simulink model "Flight3Dof_V"  (R2024b)
settings: Solver=VariableStepAuto  StartTime=0.0  StopTime=90
values from neighbouring files (symbols this model uses):
  alpha_sch = [0 0.08 0.16 0.24 0.32 0.4]    [aero_guid_autop.mat]
  Cm_q = -0.65    [aero_guid_dat.m]
  Cn_alpha = 7.609    [aero_guid_dat.m]
  Cx_fin = 0    [aero_guid_dat.m]
  Cz_fin = 5.61    [aero_guid_dat.m]
  d_ref = 0.08    [aero_guid_dat.m]
  fin_max = 35.0*d2r    (= 0.610865238198)    [aero_guid_dat.m]
  fin_min = -35.0*d2r    (= -0.610865238198)    [aero_guid_dat.m]
  g = 9.81    [aero_guid_dat.m]
  h_ini = mState(end,4)    [aero_guid_dat.m]
  K = [0.0274272658442 0.022514521532 0.0188381278441 0.0160368406712 0.0137662609944 0.0119857576445 0.0105918197111 0.00938210037551 0.00839164223299 0.0264249961464 0.0216246329404 0.0181908758086 ... (54 elements, 9x6)]    [aero_guid_autop.mat]
  Ka = [0.941240537955 0.93637246732 0.931559594469 0.926913222355 0.921953565217 0.917255055328 0.913053581223 0.908386604457 0.903975208808 0.938862932336 0.933592325749 0.928951336073 ... (54 elements, 9x6)]    [aero_guid_autop.mat]
  Kg = [0.85025548389 0.668816232249 0.539692221599 0.444760785577 0.373115794158 0.317881150033 0.273934317038 0.239434726051 0.211636994858 0.843001258735 0.661554199177 0.532424138805 ... (54 elements, 9x6)]    [aero_guid_autop.mat]
  Ki = [22.5219818693 26.1087313803 30.1256514292 34.5615685684 39.3998846557 44.6135139259 50.5273670311 56.4127258892 62.5431134445 22.709249563 26.3788303432 30.5068602639 ... (54 elements, 9x6)]    [aero_guid_autop.mat]
  l_acc = 0.07465    [aero_guid_dat.m]
  M_sch = [0 0.25 0.5 0.75 1 1.25 1.5 1.75 2]    [aero_guid_autop.mat]
  max_acc = max_load_factor*g    (= 58.86)    [aero_guid_dat.m]
  pos_tgt = [x_ini_tgt,-h_ini_tgt]    [aero_guid_dat.m]
  q_ini = 0.00001*d2r    (= 1.74532925199e-07)    [aero_guid_dat.m]
  S_ref = 0.0050    (= 0.005)    [aero_guid_dat.m]
  t_fin_burn = 30    [aero_guid_dat.m]
  theta_tgt = 180*d2r    (= 3.14159265359)    [aero_guid_dat.m]
  Thrust = 150    [aero_guid_dat.m]
  v_ini = sqrt(mState(end,1)^2+mState(end,2)^2)    [aero_guid_dat.m]
  v_tgt = 60    [aero_guid_dat.m]
  X_cp = 0.6873    [aero_guid_dat.m]
  x_ini = mState(end,3)    [aero_guid_dat.m]
undefined symbols (not defined in the file or in its folder): CG_with_time, Cx_with_M, mass_with_time, mdot, Pk_final, Pk_matrix_small, theta_vec, theta_vec_small, X_cg, X_cg_fixed_small, Y_cg, Y_cg_fixed_small
libraries: aerolibasang x3, simulink x2, aerolibanim x1, aerolibatmos2 x1, aerolibactuator x1
settings Model: Creator=vince  LastModifiedBy=vince
settings SolverCC: ZeroCrossAlgorithm=Adaptive
settings DebuggingCC: AlgebraicLoopMsg=none  IgnoredZcDiagnostic=none
settings RTWCC: GPUComputeCapability=3.5

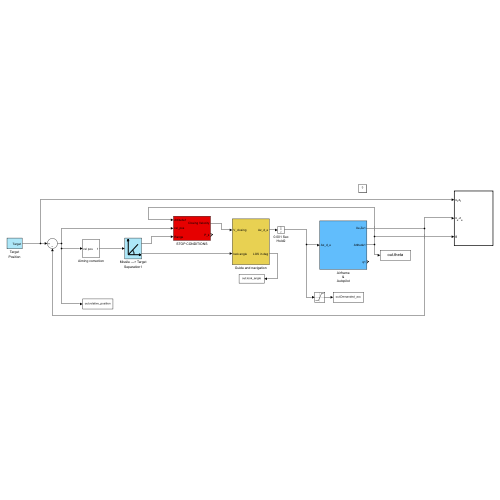
[thumbnail: Simulink's stored preview of the top-level diagram]
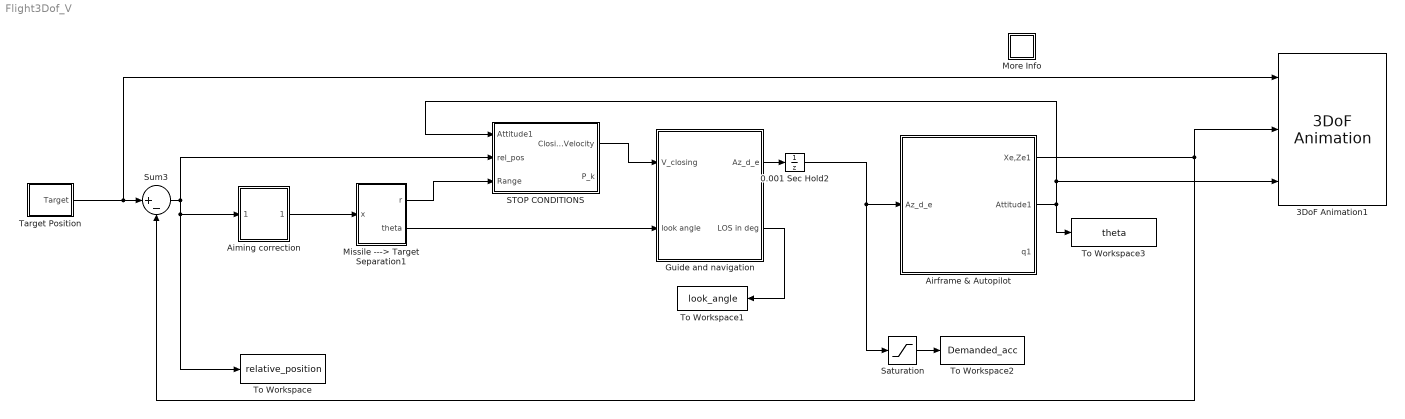
== system Flight3Dof_V ==
  0.001 Sec Hold2 : UnitDelay  SampleTime=0.001  HasFrameUpgradeWarning=on
  3DoF Animation1 : aerolibanim/3DoF Animation  u1=[0 10000 0 100000 -10000 -50]  u2=0.1  u3=5  u5=Fixed position  u6=[2000 18000 -3150]  u7=10  u8=on
  Aiming correction : Subsystem
  Airframe & Autopilot : Subsystem
  Guide and navigation : Subsystem
  Missile ---> Target Separation1 : Subsystem  mask(Cart2Polar){}
      mask help:
      | Transformation from cartesian to polar coordinates.
      | [x, y] -> [r, theta]
      |
      | r = sqrt(x^2 + y^2);
      | theta = atan(y/x);
      mask Help: Unmask this block for more help.
      mask Display: plot(0,0,100,100,[24,20,15,20,20],[85,95,85,95,20],[80,20,95,85,95,85],[70,20,20,15,20,24],[56,56,55,52,50,46],[20,26,31,35,38,42])
  More Info : Subsystem
      settings: OpenFcn=showExample('simulink_aerospace/DesigningAGuidanceSystemInMATLABAndSimulinkExample')
      mask Display: disp('?')
  STOP CONDITIONS : Subsystem
  Saturation : Saturate  UpperLimit=max_acc  LowerLimit=-max_acc
  Sum3 : Sum  Inputs=|+-  InputSameDT=on  SaturateOnIntegerOverflow=on  OutDataTypeStr=Inherit: Same as first input
  Target Position : Subsystem
  To Workspace : ToWorkspace  VariableName=relative_position  SampleTime=-1
  To Workspace1 : ToWorkspace  VariableName=look_angle  SaveFormat=Structure With Time  SampleTime=-1
  To Workspace2 : ToWorkspace  VariableName=Demanded_acc  SaveFormat=Structure With Time  SampleTime=-1
  To Workspace3 : ToWorkspace  VariableName=theta  SaveFormat=Structure With Time  SampleTime=-1
  wires:
  Sum3/1 -> To Workspace/1, Aiming correction/1(rel pos), STOP CONDITIONS/2(rel_pos)
  Target Position/1(Target) -> 3DoF Animation1/1, Sum3/1
  Airframe & Autopilot/1(Xe,Ze1) -> Sum3/2, 3DoF Animation1/2
  Airframe & Autopilot/2(Attitude1) -> To Workspace3/1, STOP CONDITIONS/1(Attitude1), 3DoF Animation1/3
  Guide and navigation/1(Az_d_e) -> 0.001 Sec Hold2/1
  Missile ---> Target Separation1/2(theta) -> Guide and navigation/2(look angle)
  Guide and navigation/2(LOS in deg) -> To Workspace1/1
  STOP CONDITIONS/1(Closing Velocity) -> Guide and navigation/1(V_closing)
  Missile ---> Target Separation1/1(r) -> STOP CONDITIONS/3(Range)
  Aiming correction/1(Out1) -> Missile ---> Target Separation1/1(x)
  0.001 Sec Hold2/1 -> Saturation/1, Airframe & Autopilot/1(Az_d_e)
  Saturation/1 -> To Workspace2/1

== system Flight3Dof_V/Aiming correction ==
  rel pos : Inport
  Add : Sum
  Add1 : Sum
  Demux1 : Demux  Outputs=2
  Mux : Mux  Inputs=2
  x error : Constant  Value=0.6
  z error : Constant  Value=0.65
  Out1 : Outport
  wires:
  rel pos/1 -> Demux1/1
  Demux1/2 -> Add1/1
  Demux1/1 -> Add/2
  Mux/1 -> Out1/1
  Add/1 -> Mux/1
  x error/1 -> Add/1
  Add1/1 -> Mux/2
  z error/1 -> Add1/2

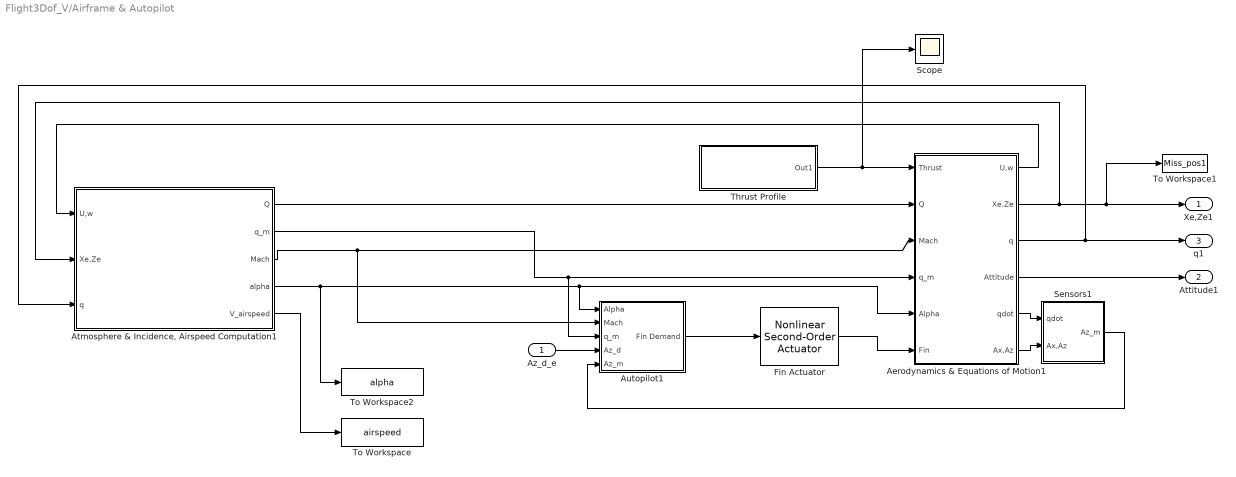
== system Flight3Dof_V/Airframe & Autopilot ==
  Az_d_e : Inport
  Aerodynamics & Equations of Motion1 : Subsystem
  "Atmosphere & Incidence, Airspeed Computation1" : Subsystem
  Autopilot1 : Subsystem
  Fin Actuator : aerolibactuator/Nonlinear Second-Order Actuator  wn_fin=wn_fin  z_fin=z_fin  fin_max=fin_max  fin_min=fin_min  fin_maxrate=fin_maxrate  fin_act_0=fin_act_0  fin_act_vel=0
  Scope : Scope
  Sensors1 : Subsystem
  Thrust Profile : Subsystem
  To Workspace : ToWorkspace  VariableName=airspeed  SaveFormat=Structure With Time  SampleTime=-1
  To Workspace1 : ToWorkspace  VariableName=Miss_pos1  SaveFormat=Structure With Time  SampleTime=-1
  To Workspace2 : ToWorkspace  VariableName=alpha  SaveFormat=Structure With Time  SampleTime=-1
  Xe,Ze1 : Outport  InitialOutput=0  VectorParamsAs1DForOutWhenUnconnected=off
  Attitude1 : Outport  Port=2  InitialOutput=0  VectorParamsAs1DForOutWhenUnconnected=off
  q1 : Outport  Port=3  InitialOutput=0  VectorParamsAs1DForOutWhenUnconnected=off
  wires:
  "Atmosphere & Incidence, Airspeed Computation1"/4(alpha) -> Autopilot1/1(Alpha), Aerodynamics & Equations of Motion1/5(Alpha), To Workspace2/1
  Aerodynamics & Equations of Motion1/3(q) -> "Atmosphere & Incidence, Airspeed Computation1"/3(q), q1/1
  "Atmosphere & Incidence, Airspeed Computation1"/2(q_m) -> Autopilot1/3(q_m), Aerodynamics & Equations of Motion1/4(q_m)
  "Atmosphere & Incidence, Airspeed Computation1"/1(Q) -> Aerodynamics & Equations of Motion1/2(Q)
  Aerodynamics & Equations of Motion1/4(Attitude) -> Attitude1/1
  Aerodynamics & Equations of Motion1/1(U,w) -> "Atmosphere & Incidence, Airspeed Computation1"/1(U,w)
  Aerodynamics & Equations of Motion1/2(Xe,Ze) -> "Atmosphere & Incidence, Airspeed Computation1"/2(Xe,Ze), To Workspace1/1, Xe,Ze1/1
  Aerodynamics & Equations of Motion1/6(Ax,Az) -> Sensors1/2(Ax,Az)
  Aerodynamics & Equations of Motion1/5(qdot) -> Sensors1/1(qdot)
  Sensors1/1(Az_m) -> Autopilot1/5(Az_m)
  "Atmosphere & Incidence, Airspeed Computation1"/3(Mach) -> Autopilot1/2(Mach), Aerodynamics & Equations of Motion1/3(Mach)
  "Atmosphere & Incidence, Airspeed Computation1"/5(V_airspeed) -> To Workspace/1
  Thrust Profile/1(Out1) -> Scope/1, Aerodynamics & Equations of Motion1/1(Thrust)
  Fin Actuator/1 -> Aerodynamics & Equations of Motion1/6(Fin)
  Az_d_e/1 -> Autopilot1/4(Az_d)
  Autopilot1/1(Fin Demand) -> Fin Actuator/1

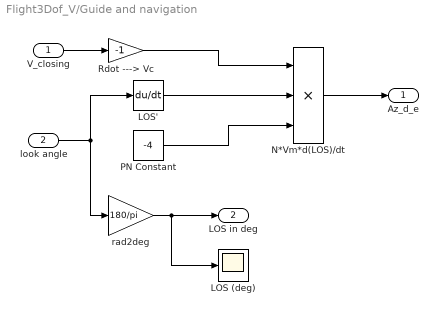
== system Flight3Dof_V/Guide and navigation ==
  V_closing : Inport
  look angle : Inport  Port=2
  LOS (deg) : Scope
  LOS' : Derivative
  N*Vm*d(LOS)/dt : Product  Inputs=3
  PN Constant : Constant  Value=-4
  Rdot ---> Vc : Gain  Gain=-1  SaturateOnIntegerOverflow=on  OutDataTypeStr=Inherit: Same as input  ParamDataTypeStr=Inherit: Same as input
  rad2deg : Gain  Gain=180/pi
  Az_d_e : Outport
  LOS in deg : Outport  Port=2
  wires:
  LOS'/1 -> N*Vm*d(LOS)/dt/2
  rad2deg/1 -> LOS (deg)/1, LOS in deg/1
  N*Vm*d(LOS)/dt/1 -> Az_d_e/1
  look angle/1 -> LOS'/1, rad2deg/1
  V_closing/1 -> Rdot ---> Vc/1
  PN Constant/1 -> N*Vm*d(LOS)/dt/3
  Rdot ---> Vc/1 -> N*Vm*d(LOS)/dt/1

== system Flight3Dof_V/Missile ---> Target Separation1 ==
  x : Inport
  Range : Fcn  Expr=hypot(u[1],u[2])
  Sightline Angle : Fcn  Expr=atan2(-u[2],u[1])
  r : Outport  InitialOutput=0  VectorParamsAs1DForOutWhenUnconnected=off
  theta : Outport  Port=2  InitialOutput=0  VectorParamsAs1DForOutWhenUnconnected=off
  wires:
  x/1 -> Sightline Angle/1, Range/1
  Range/1 -> r/1
  Sightline Angle/1 -> theta/1

== system Flight3Dof_V/More Info ==

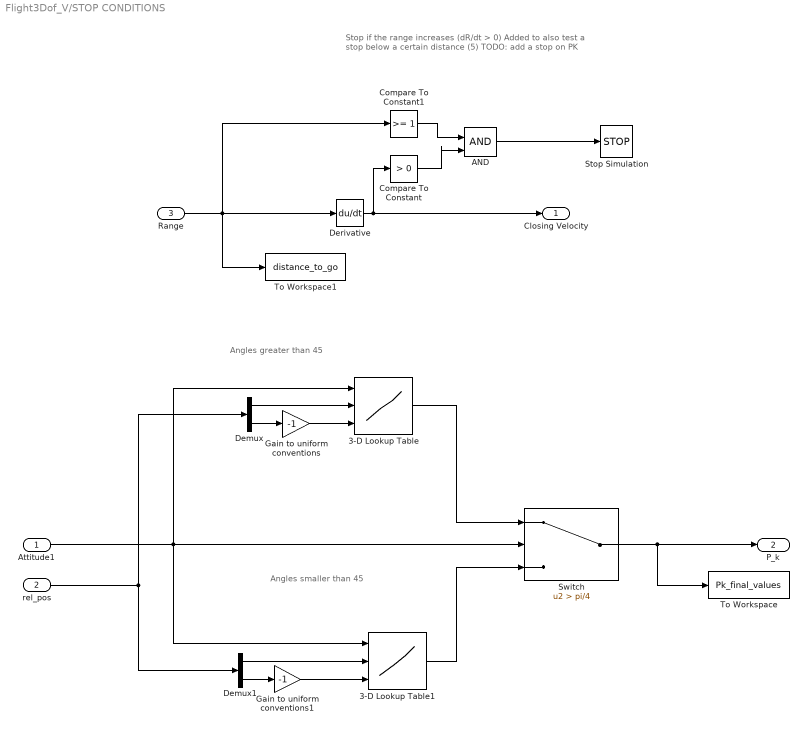
== system Flight3Dof_V/STOP CONDITIONS ==
  note: Angles greater than 45
  note: Stop if the range increases (dR/dt > 0)
      |
      | Added to also test a stop below a certain distance (5)
      |
      | TODO: add a stop on PK
  note: Angles smaller than 45
  Attitude1 : Inport
  rel_pos : Inport  Port=2
  Range : Inport  Port=3
  3-D Lookup Table : Lookup_n-D  NumberOfTableDimensions=3  BreakpointsForDimension1=theta_vec  BreakpointsForDimension2=X_cg  BreakpointsForDimension3=Y_cg  Table=Pk_final  ExtrapMethod=Clip  InternalRulePriority=Speed  RndMeth=Simplest
      settings: InputPortMap=u0,u1,u2
  3-D Lookup Table1 : Lookup_n-D  NumberOfTableDimensions=3  BreakpointsForDimension1=theta_vec_small  BreakpointsForDimension2=X_cg_fixed_small  BreakpointsForDimension3=Y_cg_fixed_small  Table=Pk_matrix_small  ExtrapMethod=Clip  InternalRulePriority=Speed  RndMeth=Simplest
      settings: InputPortMap=u0,u1,u2
  AND : Logic  IconShape=distinctive  AllPortsSameDT=off  OutDataTypeStr=boolean
  Compare To Constant : simulink/Logic and Bit Operations/Compare To Constant  relop=>  const=0  OutDataTypeStr=boolean
  Compare To Constant1 : simulink/Logic and Bit Operations/Compare To Constant  relop=>=  const=1  OutDataTypeStr=boolean
  Demux : Demux  Outputs=2
  Demux1 : Demux  Outputs=2
  Derivative : Derivative
  Gain to uniform conventions : Gain  Gain=-1
  Gain to uniform conventions1 : Gain  Gain=-1
  Stop Simulation : Stop
  Switch : Switch  Criteria=u2 > Threshold  Threshold=pi/4  SaturateOnIntegerOverflow=off  InputSameDT=off
  To Workspace : ToWorkspace  VariableName=Pk_final_values  SaveFormat=Structure With Time  SampleTime=-1
  To Workspace1 : ToWorkspace  VariableName=distance_to_go  SaveFormat=Structure With Time  SampleTime=-1
  Closing Velocity : Outport
  P_k : Outport  Port=2
  wires:
  Range/1 -> Compare To Constant1/1, Derivative/1, To Workspace1/1
  Derivative/1 -> Closing Velocity/1, Compare To Constant/1
  rel_pos/1 -> Demux/1, Demux1/1
  3-D Lookup Table/1 -> Switch/1
  Demux/1 -> 3-D Lookup Table/2
  Demux/2 -> Gain to uniform conventions/1
  Gain to uniform conventions/1 -> 3-D Lookup Table/3
  3-D Lookup Table1/1 -> Switch/3
  Demux1/2 -> Gain to uniform conventions1/1
  Demux1/1 -> 3-D Lookup Table1/2
  Attitude1/1 -> 3-D Lookup Table/1, 3-D Lookup Table1/1, Switch/2
  Gain to uniform conventions1/1 -> 3-D Lookup Table1/3
  Switch/1 -> To Workspace/1, P_k/1
  Compare To Constant1/1 -> AND/1
  Compare To Constant/1 -> AND/2
  AND/1 -> Stop Simulation/1

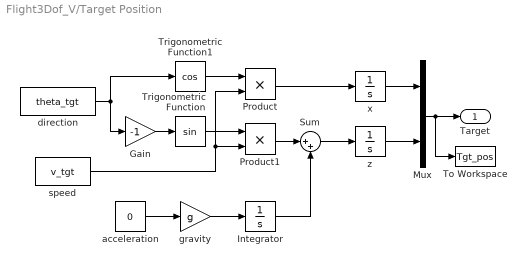
== system Flight3Dof_V/Target Position ==
  Gain : Gain  Gain=-1  SaturateOnIntegerOverflow=on  OutDataTypeStr=Inherit: Same as input  ParamDataTypeStr=Inherit: Same as input
  Integrator : Integrator
  Mux : Mux  Inputs=2
  Product : Product  InputSameDT=on  SaturateOnIntegerOverflow=on  OutDataTypeStr=Inherit: Same as first input
  Product1 : Product  InputSameDT=on  SaturateOnIntegerOverflow=on  OutDataTypeStr=Inherit: Same as first input
  Sum : Sum  Inputs=|++
  To Workspace : ToWorkspace  VariableName=Tgt_pos  SaveFormat=Structure  SampleTime=-1
  Trigonometric Function : Trigonometry
  Trigonometric Function1 : Trigonometry  Operator=cos
  acceleration : Constant  Value=0
  direction : Constant  Value=theta_tgt
  gravity : Gain  Gain=g
  speed : Constant  Value=v_tgt
  x : Integrator  InitialCondition=pos_tgt(1)
  z : Integrator  InitialCondition=pos_tgt(2)
  Target : Outport  VectorParamsAs1DForOutWhenUnconnected=off
  wires:
  x/1 -> Mux/1
  z/1 -> Mux/2
  Product/1 -> x/1
  speed/1 -> Product/2, Product1/2
  Trigonometric Function/1 -> Product1/1
  Trigonometric Function1/1 -> Product/1
  direction/1 -> Trigonometric Function1/1, Gain/1
  Gain/1 -> Trigonometric Function/1
  Mux/1 -> Target/1, To Workspace/1
  Product1/1 -> Sum/1
  Sum/1 -> z/1
  acceleration/1 -> gravity/1
  gravity/1 -> Integrator/1
  Integrator/1 -> Sum/2

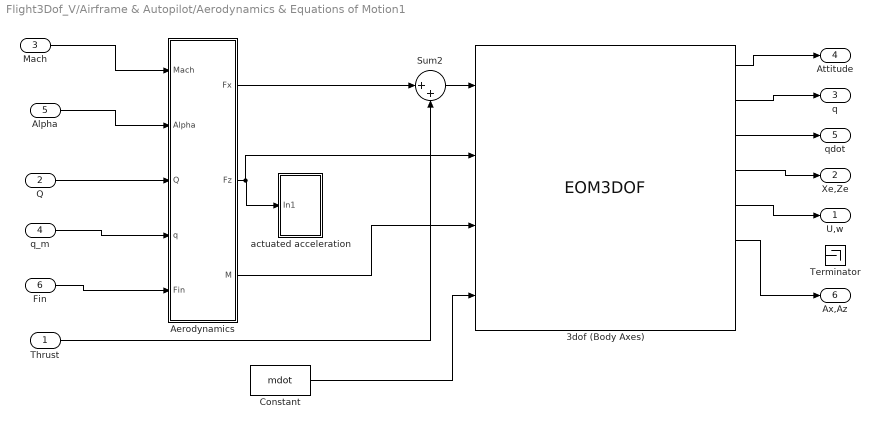
== system Flight3Dof_V/Airframe & Autopilot/Aerodynamics & Equations of Motion1 ==
  Thrust : Inport
  Q : Inport  Port=2
  Mach : Inport  Port=3
  q_m : Inport  Port=4
  Alpha : Inport  Port=5
  Fin : Inport  Port=6
  3dof (Body Axes) : EOM3DOF  mtype=Simple Variable  v_ini=v_ini  theta_ini=theta_ini  q_ini=q_ini  alpha_ini=alpha_ini  pos_ini=[x_ini -h_ini]  mass=mass_full  mass_e=mass_empty  mass_f=mass_full  Iyy=Iyy_full  Iyy_e=Iyy_empty  Iyy_f=Iyy_full  abi_flag=on
  Aerodynamics : Subsystem
  Constant : Constant  Value=mdot
  Sum2 : Sum  Inputs=|++  InputSameDT=on  SaturateOnIntegerOverflow=on  OutDataTypeStr=Inherit: Same as first input
  Terminator : Terminator
  actuated acceleration : Subsystem
  U,w : Outport  InitialOutput=0  VectorParamsAs1DForOutWhenUnconnected=off
  Xe,Ze : Outport  Port=2  InitialOutput=0  VectorParamsAs1DForOutWhenUnconnected=off
  q : Outport  Port=3  InitialOutput=0  VectorParamsAs1DForOutWhenUnconnected=off
  Attitude : Outport  Port=4  InitialOutput=0  VectorParamsAs1DForOutWhenUnconnected=off
  qdot : Outport  Port=5  InitialOutput=0  VectorParamsAs1DForOutWhenUnconnected=off
  Ax,Az : Outport  Port=6  InitialOutput=0  VectorParamsAs1DForOutWhenUnconnected=off
  wires:
  Sum2/1 -> 3dof (Body Axes)/1
  Aerodynamics/1(Fx) -> Sum2/1
  Thrust/1 -> Sum2/2
  q_m/1 -> Aerodynamics/4(q)
  Q/1 -> Aerodynamics/3(Q)
  Alpha/1 -> Aerodynamics/2(Alpha)
  3dof (Body Axes)/6 -> Ax,Az/1
  3dof (Body Axes)/5 -> U,w/1
  3dof (Body Axes)/4 -> Xe,Ze/1
  3dof (Body Axes)/3 -> qdot/1
  3dof (Body Axes)/2 -> q/1
  3dof (Body Axes)/1 -> Attitude/1
  Constant/1 -> 3dof (Body Axes)/4
  Aerodynamics/2(Fz) -> 3dof (Body Axes)/2, actuated acceleration/1(In1)
  Aerodynamics/3(" M") -> 3dof (Body Axes)/3
  Fin/1 -> Aerodynamics/5(Fin)
  Mach/1 -> Aerodynamics/1(Mach)

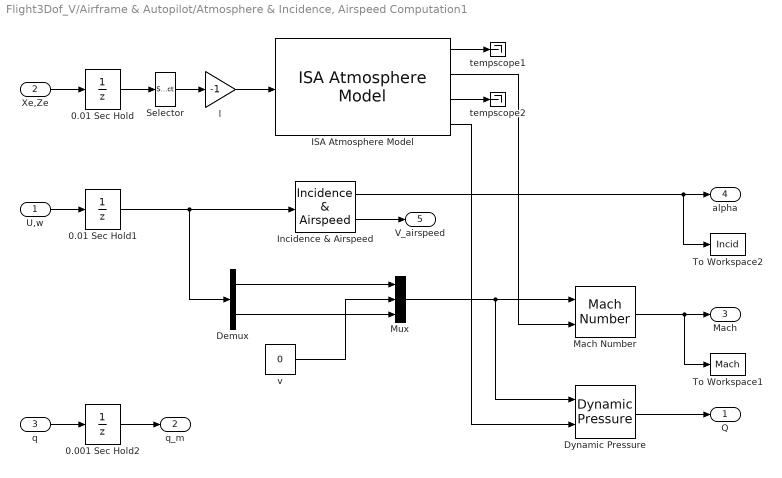
== system Flight3Dof_V/Airframe & Autopilot/Atmosphere & Incidence, Airspeed Computation1 ==
  U,w : Inport
  Xe,Ze : Inport  Port=2
  q : Inport  Port=3
  0.001 Sec Hold2 : UnitDelay  InitialCondition=q_ini  SampleTime=0.001  HasFrameUpgradeWarning=on
  0.01 Sec Hold : UnitDelay  InitialCondition=[x_ini -h_ini]  SampleTime=0.01  HasFrameUpgradeWarning=on
  0.01 Sec Hold1 : UnitDelay  InitialCondition=[v_ini 0]  SampleTime=0.01  HasFrameUpgradeWarning=on
  Demux : Demux  Outputs=2
  Dynamic Pressure : aerolibasang/Dynamic Pressure
  ISA Atmosphere Model : aerolibatmos2/ISA Atmosphere Model  useExtended=off  action=Warning  custom=off  viscosityOut=off  g=9.80665  gamma=1.4  R=287.0531  L=0.0065  h_trop=11000  h_strat=20000  rho0=1.225  P0=101325  T0=288.15  h0=0  S=110.4  Tref=273.15  muref=1.716e-5
  Incidence & Airspeed : aerolibasang/Incidence  & Airspeed
  Mach Number : aerolibasang/Mach Number
  Mux : Mux  Inputs=3
  Selector : Selector  InputPortWidth=2  IndexOptions=Index vector (dialog)  Indices=[2]  OutputSizes=1
  To Workspace1 : ToWorkspace  VariableName=Mach  SaveFormat=Structure With Time  SampleTime=-1
  To Workspace2 : ToWorkspace  VariableName=Incid  SaveFormat=Structure With Time  SampleTime=-1
  l : Gain  Gain=-1  SaturateOnIntegerOverflow=on  OutDataTypeStr=Inherit: Same as input  ParamDataTypeStr=Inherit: Same as input
  tempscope1 : Terminator
  tempscope2 : Terminator
  v : Constant  Value=0
  Q : Outport
  q_m : Outport  Port=2
  Mach : Outport  Port=3
  alpha : Outport  Port=4
  V_airspeed : Outport  Port=5
  wires:
  U,w/1 -> 0.01 Sec Hold1/1
  Incidence & Airspeed/1 -> To Workspace2/1, alpha/1
  Demux/1 -> Mux/1
  Demux/2 -> Mux/3
  v/1 -> Mux/2
  Mux/1 -> Mach Number/1, Dynamic Pressure/1
  Incidence & Airspeed/2 -> V_airspeed/1
  ISA Atmosphere Model/4 -> Dynamic Pressure/2
  Mach Number/1 -> To Workspace1/1, Mach/1
  Dynamic Pressure/1 -> Q/1
  0.01 Sec Hold1/1 -> Incidence & Airspeed/1, Demux/1
  0.01 Sec Hold/1 -> Selector/1
  l/1 -> ISA Atmosphere Model/1
  ISA Atmosphere Model/1 -> tempscope1/1
  ISA Atmosphere Model/3 -> tempscope2/1
  Selector/1 -> l/1
  Xe,Ze/1 -> 0.01 Sec Hold/1
  ISA Atmosphere Model/2 -> Mach Number/2
  0.001 Sec Hold2/1 -> q_m/1
  q/1 -> 0.001 Sec Hold2/1

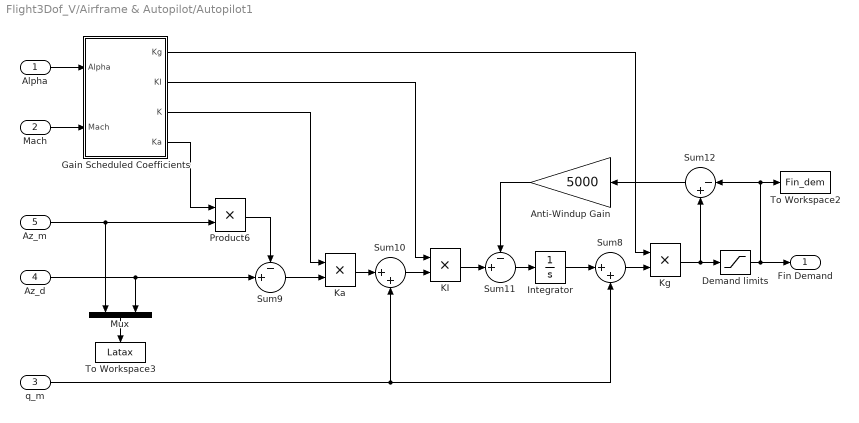
== system Flight3Dof_V/Airframe & Autopilot/Autopilot1 ==
  Alpha : Inport
  Mach : Inport  Port=2
  q_m : Inport  Port=3
  Az_d : Inport  Port=4
  Az_m : Inport  Port=5
  Anti-Windup Gain : Gain  Gain=5000  SaturateOnIntegerOverflow=on  OutDataTypeStr=Inherit: Same as input  ParamDataTypeStr=Inherit: Same as input
  "Demand limits " : Saturate  UpperLimit=fin_max  LowerLimit=fin_min
  Gain Scheduled Coefficients : Subsystem
  Integrator : Integrator
  KI : Product  InputSameDT=on  SaturateOnIntegerOverflow=on  OutDataTypeStr=Inherit: Same as first input
  Ka : Product  InputSameDT=on  SaturateOnIntegerOverflow=on  OutDataTypeStr=Inherit: Same as first input
  Kg : Product  InputSameDT=on  SaturateOnIntegerOverflow=on  OutDataTypeStr=Inherit: Same as first input
  Mux : Mux  Inputs=2
  Product6 : Product  InputSameDT=on  SaturateOnIntegerOverflow=on  OutDataTypeStr=Inherit: Same as first input
  Sum10 : Sum  Inputs=|++  InputSameDT=on  SaturateOnIntegerOverflow=on  OutDataTypeStr=Inherit: Same as first input
  Sum11 : Sum  Inputs=-+|  InputSameDT=on  SaturateOnIntegerOverflow=on  OutDataTypeStr=Inherit: Same as first input
  Sum12 : Sum  Inputs=|-+  InputSameDT=on  SaturateOnIntegerOverflow=on  OutDataTypeStr=Inherit: Same as first input
  Sum8 : Sum  Inputs=|++  InputSameDT=on  SaturateOnIntegerOverflow=on  OutDataTypeStr=Inherit: Same as first input
  Sum9 : Sum  Inputs=-+|  InputSameDT=on  SaturateOnIntegerOverflow=on  OutDataTypeStr=Inherit: Same as first input
  To Workspace2 : ToWorkspace  VariableName=Fin_dem  SaveFormat=Structure With Time  SampleTime=-1
  To Workspace3 : ToWorkspace  VariableName=Latax  SaveFormat=Structure With Time  SampleTime=-1
  Fin Demand : Outport  InitialOutput=0  VectorParamsAs1DForOutWhenUnconnected=off
  wires:
  Mach/1 -> Gain Scheduled Coefficients/2(Mach)
  Alpha/1 -> Gain Scheduled Coefficients/1(Alpha)
  Kg/1 -> Sum12/2, "Demand limits "/1
  Gain Scheduled Coefficients/1("Kg ") -> Kg/1
  Gain Scheduled Coefficients/3("K ") -> Ka/1
  Gain Scheduled Coefficients/2("KI ") -> KI/1
  Anti-Windup Gain/1 -> Sum11/1
  Sum8/1 -> Kg/2
  Integrator/1 -> Sum8/1
  Sum11/1 -> Integrator/1
  Product6/1 -> Sum9/1
  Sum9/1 -> Ka/2
  Ka/1 -> Sum10/1
  Sum10/1 -> KI/2
  KI/1 -> Sum11/2
  Sum12/1 -> Anti-Windup Gain/1
  Az_d/1 -> Mux/2, Sum9/2
  Mux/1 -> To Workspace3/1
  q_m/1 -> Sum10/2, Sum8/2
  "Demand limits "/1 -> Fin Demand/1, Sum12/1, To Workspace2/1
  Az_m/1 -> Mux/1, Product6/2
  Gain Scheduled Coefficients/4("Ka ") -> Product6/1

== system Flight3Dof_V/Airframe & Autopilot/Sensors1 ==
  qdot : Inport
  Ax,Az : Inport  Port=2
  Selector : Selector  InputPortWidth=2  IndexOptions=Index vector (dialog)  Indices=[2]  OutputSizes=1
  Sum : Sum  Inputs=-+|  InputSameDT=on  SaturateOnIntegerOverflow=on  OutDataTypeStr=Inherit: Same as first input
  l : Gain  Gain=l_acc  SaturateOnIntegerOverflow=on  OutDataTypeStr=Inherit: Same as input  ParamDataTypeStr=Inherit: Same as input
  Az_m : Outport  InitialOutput=0  VectorParamsAs1DForOutWhenUnconnected=off
  wires:
  Selector/1 -> Sum/2
  Ax,Az/1 -> Selector/1
  l/1 -> Sum/1
  Sum/1 -> Az_m/1  "Accelerometer"
  qdot/1 -> l/1

== system Flight3Dof_V/Airframe & Autopilot/Thrust Profile ==
  Clock1 : Clock
  Constant : Constant  Value=0
  Scope : Scope
  Switch : Switch  Criteria=u2 > Threshold  Threshold=t_fin_burn  SaturateOnIntegerOverflow=off  InputSameDT=off
  Thrust : Constant  Value=Thrust
  Out1 : Outport
  wires:
  Thrust/1 -> Switch/3
  Constant/1 -> Switch/1
  Switch/1 -> Scope/1, Out1/1
  Clock1/1 -> Switch/2

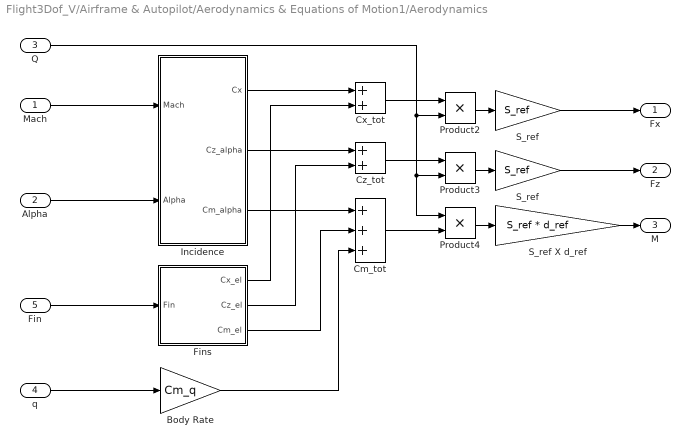
== system Flight3Dof_V/Airframe & Autopilot/Aerodynamics & Equations of Motion1/Aerodynamics ==
  Mach : Inport
  Alpha : Inport  Port=2
  Q : Inport  Port=3
  q : Inport  Port=4
  Fin : Inport  Port=5
  Body Rate : Gain  Gain=Cm_q  SaturateOnIntegerOverflow=on  OutDataTypeStr=Inherit: Same as input  ParamDataTypeStr=Inherit: Same as input
  Cm_tot : Sum  Inputs=+++  InputSameDT=on  SaturateOnIntegerOverflow=on  OutDataTypeStr=Inherit: Same as first input
  Cx_tot : Sum  InputSameDT=on  SaturateOnIntegerOverflow=on  OutDataTypeStr=Inherit: Same as first input
  Cz_tot : Sum  InputSameDT=on  SaturateOnIntegerOverflow=on  OutDataTypeStr=Inherit: Same as first input
  Fins : Subsystem
  Incidence : Subsystem
  Product2 : Product  InputSameDT=on  SaturateOnIntegerOverflow=on  OutDataTypeStr=Inherit: Same as first input
  Product3 : Product  InputSameDT=on  SaturateOnIntegerOverflow=on  OutDataTypeStr=Inherit: Same as first input
  Product4 : Product  InputSameDT=on  SaturateOnIntegerOverflow=on  OutDataTypeStr=Inherit: Same as first input
  S_ref : Gain  Gain=S_ref  SaturateOnIntegerOverflow=on  OutDataTypeStr=Inherit: Same as input  ParamDataTypeStr=Inherit: Same as input
  "S_ref " : Gain  Gain=S_ref  SaturateOnIntegerOverflow=on  OutDataTypeStr=Inherit: Same as input  ParamDataTypeStr=Inherit: Same as input
  S_ref X d_ref : Gain  Gain=S_ref * d_ref  SaturateOnIntegerOverflow=on  OutDataTypeStr=Inherit: Same as input  ParamDataTypeStr=Inherit: Same as input
  Fx : Outport  InitialOutput=[0]  VectorParamsAs1DForOutWhenUnconnected=off
  Fz : Outport  Port=2  InitialOutput=0  VectorParamsAs1DForOutWhenUnconnected=off
  " M" : Outport  Port=3  InitialOutput=0  VectorParamsAs1DForOutWhenUnconnected=off
  wires:
  Incidence/1(Cx) -> Cx_tot/1
  Fins/1(Cx_el) -> Cx_tot/2
  Incidence/2(Cz_alpha) -> Cz_tot/1
  Fins/2(Cz_el) -> Cz_tot/2
  Incidence/3(Cm_alpha) -> Cm_tot/1
  Fins/3(Cm_el) -> Cm_tot/2
  Body Rate/1 -> Cm_tot/3
  Alpha/1 -> Incidence/2(Alpha)
  Cx_tot/1 -> Product2/1
  Cz_tot/1 -> Product3/1
  Product2/1 -> S_ref/1
  S_ref/1 -> Fx/1
  Product3/1 -> "S_ref "/1
  "S_ref "/1 -> Fz/1
  S_ref X d_ref/1 -> " M"/1
  Product4/1 -> S_ref X d_ref/1
  Cm_tot/1 -> Product4/2
  q/1 -> Body Rate/1
  Q/1 -> Product4/1, Product3/2, Product2/2
  Fin/1 -> Fins/1(Fin)
  Mach/1 -> Incidence/1(Mach)

== system Flight3Dof_V/Airframe & Autopilot/Aerodynamics & Equations of Motion1/actuated acceleration ==
  note: X ANTONIO:
      |  Add this to the plot
  note: The applied force is divided by the mass at time t to study the actuated acceleration.
  In1 : Inport
  1-D Lookup Table : Lookup_n-D  NumberOfTableDimensions=1  BreakpointsForDimension1=mass_with_time(1,:)  Table=mass_with_time(2,:)  ExtrapMethod=Clip  InternalRulePriority=Speed  RndMeth=Simplest
  Clock : Clock
  Divide : Product  Inputs=*/
  Scope : Scope
  To Workspace : ToWorkspace  VariableName=Actuated_acc  SaveFormat=Structure With Time  SampleTime=-1
  wires:
  Divide/1 -> To Workspace/1, Scope/1
  In1/1 -> Divide/1
  Clock/1 -> 1-D Lookup Table/1
  1-D Lookup Table/1 -> Divide/2

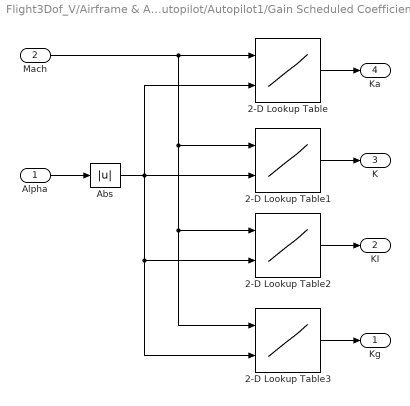
== system Flight3Dof_V/Airframe & Autopilot/Autopilot1/Gain Scheduled Coefficients ==
  Alpha : Inport
  Mach : Inport  Port=2
  2-D Lookup Table : Lookup_n-D  BreakpointsForDimension1=M_sch  BreakpointsForDimension2=alpha_sch  Table=Ka  InternalRulePriority=Speed  RndMeth=Simplest
      settings: InputPortMap=u0,u1
  2-D Lookup Table1 : Lookup_n-D  BreakpointsForDimension1=M_sch  BreakpointsForDimension2=alpha_sch  Table=K  InternalRulePriority=Speed  RndMeth=Simplest
      settings: InputPortMap=u0,u1
  2-D Lookup Table2 : Lookup_n-D  BreakpointsForDimension1=M_sch  BreakpointsForDimension2=alpha_sch  Table=Ki  InternalRulePriority=Speed  RndMeth=Simplest
      settings: InputPortMap=u0,u1
  2-D Lookup Table3 : Lookup_n-D  BreakpointsForDimension1=M_sch  BreakpointsForDimension2=alpha_sch  Table=Kg  InternalRulePriority=Speed  RndMeth=Simplest
      settings: InputPortMap=u0,u1
  Abs : Abs
  "Kg " : Outport  InitialOutput=0  VectorParamsAs1DForOutWhenUnconnected=off
  "KI " : Outport  Port=2  InitialOutput=0  VectorParamsAs1DForOutWhenUnconnected=off
  "K " : Outport  Port=3  InitialOutput=0  VectorParamsAs1DForOutWhenUnconnected=off
  "Ka " : Outport  Port=4  InitialOutput=0  VectorParamsAs1DForOutWhenUnconnected=off
  wires:
  Alpha/1 -> Abs/1
  2-D Lookup Table/1 -> "Ka "/1
  2-D Lookup Table1/1 -> "K "/1
  2-D Lookup Table2/1 -> "KI "/1
  2-D Lookup Table3/1 -> "Kg "/1
  Mach/1 -> 2-D Lookup Table3/1, 2-D Lookup Table2/1, 2-D Lookup Table1/1, 2-D Lookup Table/1
  Abs/1 -> 2-D Lookup Table3/2, 2-D Lookup Table2/2, 2-D Lookup Table/2, 2-D Lookup Table1/2

== system Flight3Dof_V/Airframe & Autopilot/Aerodynamics & Equations of Motion1/Aerodynamics/Fins ==
  Fin : Inport
  Cm_fin : Subsystem
  Cx : Gain  Gain=Cx_fin  SaturateOnIntegerOverflow=on  OutDataTypeStr=Inherit: Same as input  ParamDataTypeStr=Inherit: Same as input
  Cz : Gain  Gain=Cz_fin  SaturateOnIntegerOverflow=on  OutDataTypeStr=Inherit: Same as input  ParamDataTypeStr=Inherit: Same as input
  Cx_el : Outport  InitialOutput=0  VectorParamsAs1DForOutWhenUnconnected=off
  Cz_el : Outport  Port=2  InitialOutput=0  VectorParamsAs1DForOutWhenUnconnected=off
  Cm_el : Outport  Port=3  InitialOutput=0  VectorParamsAs1DForOutWhenUnconnected=off
  wires:
  Fin/1 -> Cm_fin/1(Fin), Cz/1, Cx/1
  Cx/1 -> Cx_el/1
  Cz/1 -> Cz_el/1
  Cm_fin/1(Cm_el) -> Cm_el/1

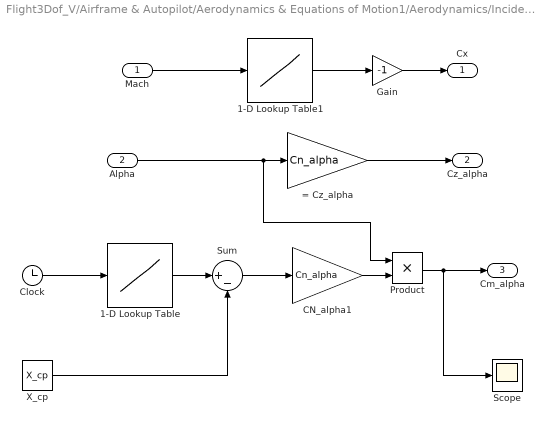
== system Flight3Dof_V/Airframe & Autopilot/Aerodynamics & Equations of Motion1/Aerodynamics/Incidence ==
  Mach : Inport
  Alpha : Inport  Port=2
  1-D Lookup Table : Lookup_n-D  NumberOfTableDimensions=1  BreakpointsForDimension1=CG_with_time(1,:)  Table=CG_with_time(2,:)  ExtrapMethod=Clip  InternalRulePriority=Speed  RndMeth=Simplest
  1-D Lookup Table1 : Lookup_n-D  NumberOfTableDimensions=1  BreakpointsForDimension1=Cx_with_M(2,:)  Table=Cx_with_M(1,:)  ExtrapMethod=Clip  InternalRulePriority=Speed  RndMeth=Simplest
  = Cz_alpha : Gain  Gain=Cn_alpha
  CN_alpha1 : Gain  Gain=Cn_alpha
  Clock : Clock
  Gain : Gain  Gain=-1
  Product : Product
  Scope : Scope
  Sum : Sum  Inputs=|+-
  X_cp : Constant  Value=X_cp
  Cx : Outport  InitialOutput=0  VectorParamsAs1DForOutWhenUnconnected=off
  Cz_alpha : Outport  Port=2  InitialOutput=0  VectorParamsAs1DForOutWhenUnconnected=off
  Cm_alpha : Outport  Port=3  InitialOutput=0  VectorParamsAs1DForOutWhenUnconnected=off
  wires:
  Alpha/1 -> Product/1, = Cz_alpha/1
  = Cz_alpha/1 -> Cz_alpha/1
  CN_alpha1/1 -> Product/2
  Sum/1 -> CN_alpha1/1
  X_cp/1 -> Sum/2
  Product/1 -> Scope/1, Cm_alpha/1
  1-D Lookup Table/1 -> Sum/1
  Clock/1 -> 1-D Lookup Table/1
  Mach/1 -> 1-D Lookup Table1/1
  1-D Lookup Table1/1 -> Gain/1
  Gain/1 -> Cx/1

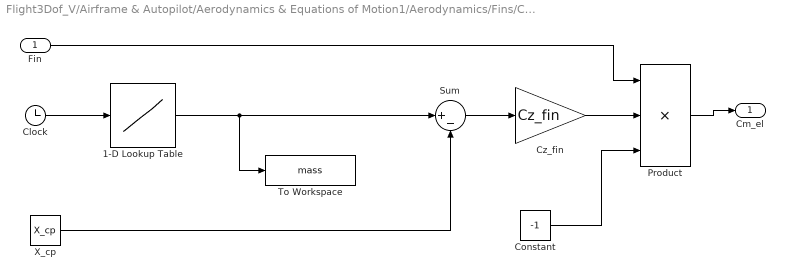
== system Flight3Dof_V/Airframe & Autopilot/Aerodynamics & Equations of Motion1/Aerodynamics/Fins/Cm_fin ==
  Fin : Inport
  1-D Lookup Table : Lookup_n-D  NumberOfTableDimensions=1  BreakpointsForDimension1=CG_with_time(1,:)  Table=CG_with_time(2,:)  ExtrapMethod=Clip  InternalRulePriority=Speed  RndMeth=Simplest
  Clock : Clock
  Constant : Constant  Value=-1
  Cz_fin : Gain  Gain=Cz_fin
  Product : Product  Inputs=3
  Sum : Sum  Inputs=|+-
  To Workspace : ToWorkspace  VariableName=mass  SaveFormat=Structure With Time  SampleTime=-1
  X_cp : Constant  Value=X_cp
  Cm_el : Outport
  wires:
  Clock/1 -> 1-D Lookup Table/1
  X_cp/1 -> Sum/2
  Sum/1 -> Cz_fin/1
  Cz_fin/1 -> Product/2
  Product/1 -> Cm_el/1
  Fin/1 -> Product/1
  1-D Lookup Table/1 -> To Workspace/1, Sum/1
  Constant/1 -> Product/3
